simulink model "RF_Digital_Twin_Demo"  (R2025a)
settings: Solver=VariableStepAuto  StartTime=0.0  StopTime=10.0  RelTol=1e-3
values from neighbouring files (symbols this model uses):
  classes5 = {'AM-DSB','BPSK','QAM16','QPSK','WBFM'}    [AI_Training.m]
  net1D = trainNetwork(XTrainSeq,YTrainCNN,layers1D,options1D)    [AI_Training.m]
undefined symbols (not defined in the file or in its folder): classify, modulation, snr, X
settings Model: Creator=saisa  LastModifiedBy=saisa

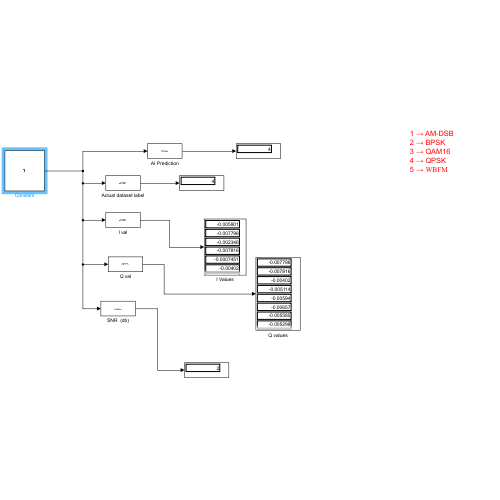
[thumbnail: Simulink's stored preview of the top-level diagram]
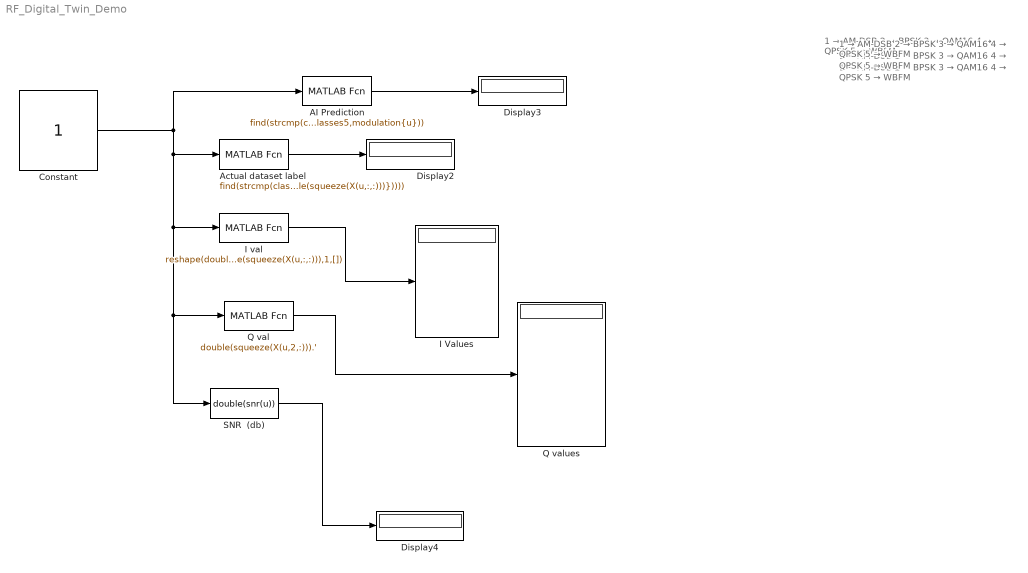
== system RF_Digital_Twin_Demo ==
  note: 1 → AM-DSB
      | 2 → BPSK
      | 3 → QAM16
      | 4 → QPSK
      | 5 → WBFM
  note: 1 → AM-DSB
      | 2 → BPSK
      | 3 → QAM16
      | 4 → QPSK
      | 5 → WBFM
  note: 1 → AM-DSB
      | 2 → BPSK
      | 3 → QAM16
      | 4 → QPSK
      | 5 → WBFM
  note: 1 → AM-DSB
      | 2 → BPSK
      | 3 → QAM16
      | 4 → QPSK
      | 5 → WBFM
  AI Prediction : MATLABFcn  MATLABFcn=find(strcmp(classes5,modulation{u}))  OutputDimensions=1
  Actual dataset label : MATLABFcn  MATLABFcn=find(strcmp(classes5,char(classify(net1D,{double(squeeze(X(u,:,:)))}))))  OutputDimensions=1
  Constant : Constant
  Display2 : Display
  Display3 : Display
  Display4 : Display
  I Values : Display
  I val : MATLABFcn  MATLABFcn=reshape(double(squeeze(X(u,:,:))),1,[])  OutputDimensions=256
  Q val : MATLABFcn  MATLABFcn=double(squeeze(X(u,2,:))).'  OutputDimensions=128
  Q values : Display
  SNR  (db) : MATLABFcn  MATLABFcn=double(snr(u))  OutputDimensions=1
  wires:
  Constant/1 -> Actual dataset label/1, I val/1, SNR  (db)/1, Q val/1, AI Prediction/1
  I val/1 -> I Values/1
  Q val/1 -> Q values/1
  Actual dataset label/1 -> Display2/1
  SNR  (db)/1 -> Display4/1
  AI Prediction/1 -> Display3/1
